simulink model "pmsm_mechanical_bench"  (R2024b)
settings: Solver=ode4  StartTime=0.0  StopTime=bench.StopTime  FixedStep=bench.SolverStep  RelTol=1e-3
model workspace (MAT data in the model file):
  bench.J = 0.002
  bench.B = 0.001
  bench.Tc = 0.02
  bench.FrictionSpeed = 0.2
  bench.QuadraticFriction = 0
  bench.PolePairs = 3
  bench.Flux = 0.03
  bench.Ld = 0.004
  bench.Lq = 0.006
  bench.CurrentTimeConstant = 0.002
  bench.SpeedLoopEnabled = 1
  bench.Kp = 0.2
  bench.Ki = 0.3
  bench.CurrentLimit = 6
  bench.InitialPI = 0
  bench.InitialId = 0
  bench.InitialIq = 0
  bench.InitialSpeed = 35
  bench.SolverStep = 0.0001
  bench.SamplePeriod = 0.001
  bench.StopTime = 3
values from neighbouring files (symbols this model uses):
  bench = struct('Rs',0.7,'Ld',0.004,'Lq',0.006,'Flux',0.03,      'VoltageDrop',0.35,'ResistanceDrop',0.03,'ZeroCurrent',0.15,      'Phase',0,'StopTime',0.6,'SolverStep',1e-5,'SamplePeriod',1e-4,      'InitialDCurrent',0,'InitialQCurrent',0,      'DVoltageBias',1.2,'DVoltageAmplitude',[0.8,0.35],      'DVoltageFrequency',[31,9],'QVoltageBias',5,      'QVoltageAmplitude',[1.1,0.6],'QVoltageFrequency',[17,4], ...(+61 chars)    [pmsm_bench_defaults.m]    (also in pmsm_mechanical_defaults.m = struct('J',0.002,'B',0.001,'Tc',0.02,'FrictionSpeed',0.2,   ; pmsm_run_mechanical_benchmark.m = pmsm_mechanical_defaults(); pmsm_run_simulink_benchmark.m = pmsm_bench_defaults())
settings Model: Creator=lxy  LastModifiedBy=lxy

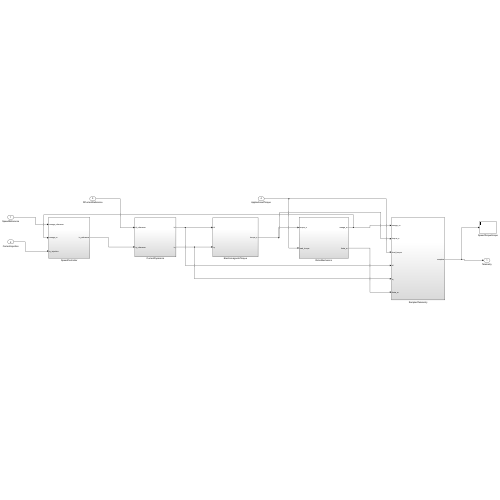
[thumbnail: Simulink's stored preview of the top-level diagram]
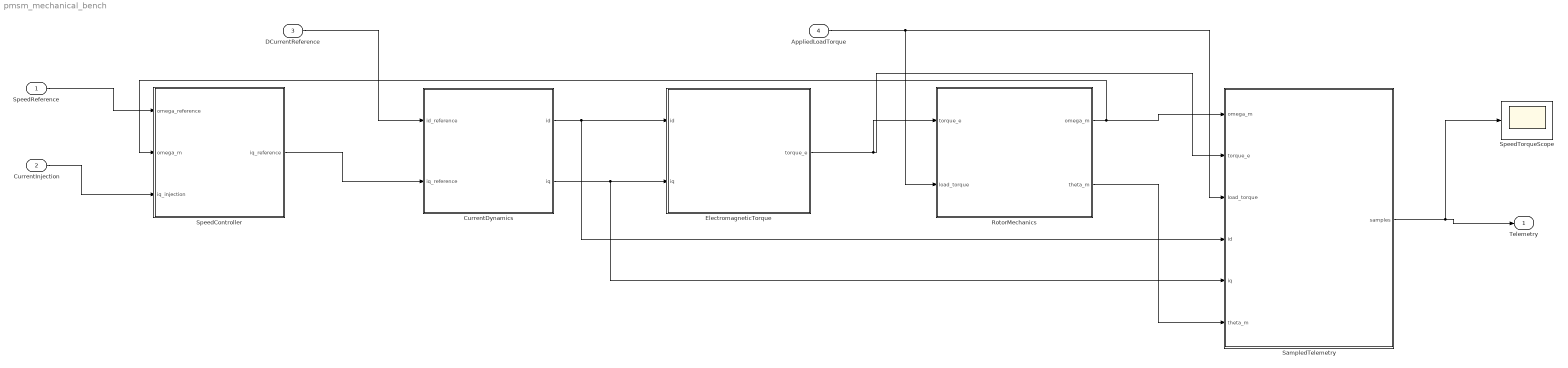
== system pmsm_mechanical_bench ==
  SpeedReference : Inport
  CurrentInjection : Inport  Port=2
  DCurrentReference : Inport  Port=3
  AppliedLoadTorque : Inport  Port=4
  CurrentDynamics : Subsystem
  ElectromagneticTorque : Subsystem
  RotorMechanics : Subsystem
  SampledTelemetry : Subsystem
  SpeedController : Subsystem
  SpeedTorqueScope : Scope
  Telemetry : Outport
  wires:
  SampledTelemetry/1(samples) -> SpeedTorqueScope/1, Telemetry/1
  RotorMechanics/2(theta_m) -> SampledTelemetry/6(theta_m)
  AppliedLoadTorque/1 -> RotorMechanics/2(load_torque), SampledTelemetry/3(load_torque)
  ElectromagneticTorque/1(torque_e) -> SampledTelemetry/2(torque_e), RotorMechanics/1(torque_e)
  CurrentDynamics/2(iq) -> ElectromagneticTorque/2(iq), SampledTelemetry/5(iq)
  CurrentDynamics/1(id) -> ElectromagneticTorque/1(id), SampledTelemetry/4(id)
  SpeedController/1(iq_reference) -> CurrentDynamics/2(iq_reference)
  DCurrentReference/1 -> CurrentDynamics/1(id_reference)
  CurrentInjection/1 -> SpeedController/3(iq_injection)
  RotorMechanics/1(omega_m) -> SpeedController/2(omega_m), SampledTelemetry/1(omega_m)
  SpeedReference/1 -> SpeedController/1(omega_reference)

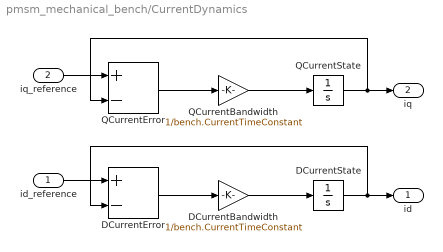
== system pmsm_mechanical_bench/CurrentDynamics ==
  id_reference : Inport
  iq_reference : Inport  Port=2
  DCurrentBandwidth : Gain  Gain=1/bench.CurrentTimeConstant
  DCurrentError : Sum  Inputs=+-
  DCurrentState : Integrator  InitialCondition=bench.InitialId
  QCurrentBandwidth : Gain  Gain=1/bench.CurrentTimeConstant
  QCurrentError : Sum  Inputs=+-
  QCurrentState : Integrator  InitialCondition=bench.InitialIq
  id : Outport
  iq : Outport  Port=2
  wires:
  QCurrentBandwidth/1 -> QCurrentState/1
  QCurrentError/1 -> QCurrentBandwidth/1
  QCurrentState/1 -> QCurrentError/2, iq/1
  iq_reference/1 -> QCurrentError/1
  DCurrentBandwidth/1 -> DCurrentState/1
  DCurrentError/1 -> DCurrentBandwidth/1
  DCurrentState/1 -> DCurrentError/2, id/1
  id_reference/1 -> DCurrentError/1

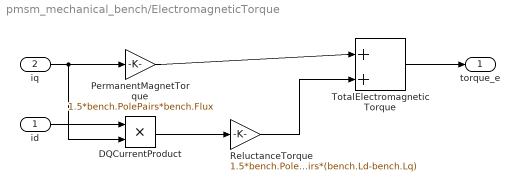
== system pmsm_mechanical_bench/ElectromagneticTorque ==
  id : Inport
  iq : Inport  Port=2
  DQCurrentProduct : Product  Inputs=**
  PermanentMagnetTorque : Gain  Gain=1.5*bench.PolePairs*bench.Flux
  ReluctanceTorque : Gain  Gain=1.5*bench.PolePairs*(bench.Ld-bench.Lq)
  TotalElectromagneticTorque : Sum  Inputs=|++
  torque_e : Outport
  wires:
  TotalElectromagneticTorque/1 -> torque_e/1
  ReluctanceTorque/1 -> TotalElectromagneticTorque/2
  PermanentMagnetTorque/1 -> TotalElectromagneticTorque/1
  DQCurrentProduct/1 -> ReluctanceTorque/1
  id/1 -> DQCurrentProduct/1
  iq/1 -> PermanentMagnetTorque/1, DQCurrentProduct/2

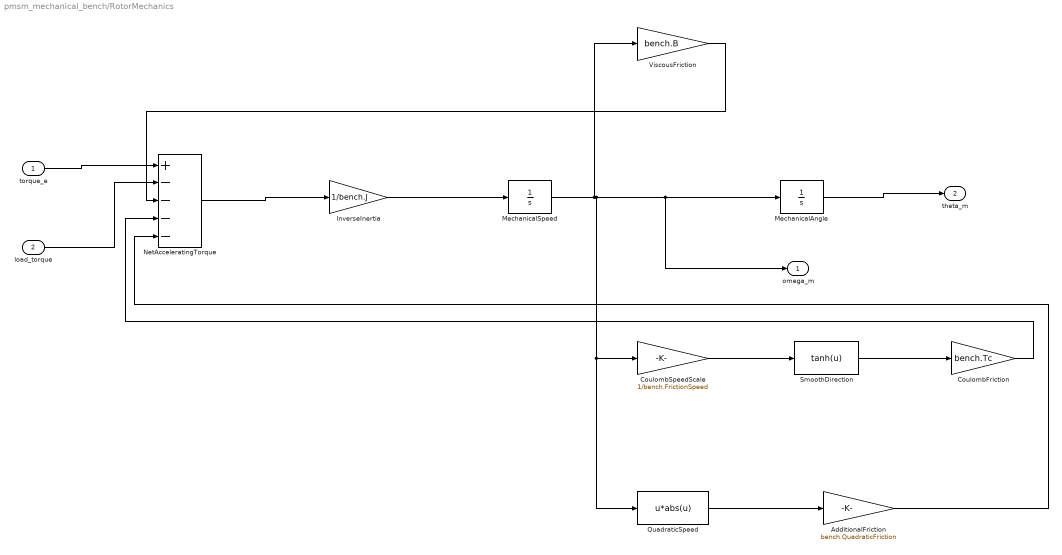
== system pmsm_mechanical_bench/RotorMechanics ==
  torque_e : Inport
  load_torque : Inport  Port=2
  AdditionalFriction : Gain  Gain=bench.QuadraticFriction
  CoulombFriction : Gain  Gain=bench.Tc
  CoulombSpeedScale : Gain  Gain=1/bench.FrictionSpeed
  InverseInertia : Gain  Gain=1/bench.J
  MechanicalAngle : Integrator
  MechanicalSpeed : Integrator  InitialCondition=bench.InitialSpeed
  NetAcceleratingTorque : Sum  Inputs=+----
  QuadraticSpeed : Fcn  Expr=u*abs(u)
  SmoothDirection : Fcn  Expr=tanh(u)
  ViscousFriction : Gain  Gain=bench.B
  omega_m : Outport
  theta_m : Outport  Port=2
  wires:
  MechanicalAngle/1 -> theta_m/1
  QuadraticSpeed/1 -> AdditionalFriction/1
  SmoothDirection/1 -> CoulombFriction/1
  CoulombSpeedScale/1 -> SmoothDirection/1
  MechanicalSpeed/1 -> CoulombSpeedScale/1, QuadraticSpeed/1, omega_m/1, MechanicalAngle/1, ViscousFriction/1
  InverseInertia/1 -> MechanicalSpeed/1
  NetAcceleratingTorque/1 -> InverseInertia/1
  AdditionalFriction/1 -> NetAcceleratingTorque/5
  CoulombFriction/1 -> NetAcceleratingTorque/4
  ViscousFriction/1 -> NetAcceleratingTorque/3
  load_torque/1 -> NetAcceleratingTorque/2
  torque_e/1 -> NetAcceleratingTorque/1

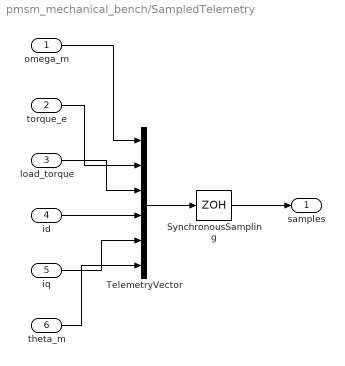
== system pmsm_mechanical_bench/SampledTelemetry ==
  omega_m : Inport
  torque_e : Inport  Port=2
  load_torque : Inport  Port=3
  id : Inport  Port=4
  iq : Inport  Port=5
  theta_m : Inport  Port=6
  SynchronousSampling : ZeroOrderHold  SampleTime=bench.SamplePeriod
  TelemetryVector : Mux  Inputs=6
  samples : Outport
  wires:
  SynchronousSampling/1 -> samples/1
  TelemetryVector/1 -> SynchronousSampling/1
  theta_m/1 -> TelemetryVector/6
  iq/1 -> TelemetryVector/5
  id/1 -> TelemetryVector/4
  load_torque/1 -> TelemetryVector/3
  torque_e/1 -> TelemetryVector/2
  omega_m/1 -> TelemetryVector/1

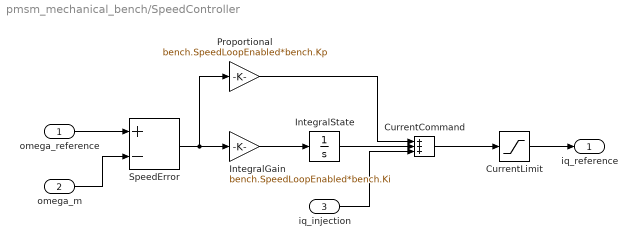
== system pmsm_mechanical_bench/SpeedController ==
  omega_reference : Inport
  omega_m : Inport  Port=2
  iq_injection : Inport  Port=3
  CurrentCommand : Sum  Inputs=+++
  CurrentLimit : Saturate  UpperLimit=bench.CurrentLimit  LowerLimit=-bench.CurrentLimit
  IntegralGain : Gain  Gain=bench.SpeedLoopEnabled*bench.Ki
  IntegralState : Integrator  InitialCondition=bench.InitialPI
  Proportional : Gain  Gain=bench.SpeedLoopEnabled*bench.Kp
  SpeedError : Sum  Inputs=+-
  iq_reference : Outport
  wires:
  CurrentLimit/1 -> iq_reference/1
  CurrentCommand/1 -> CurrentLimit/1
  iq_injection/1 -> CurrentCommand/3
  IntegralState/1 -> CurrentCommand/2
  Proportional/1 -> CurrentCommand/1
  IntegralGain/1 -> IntegralState/1
  SpeedError/1 -> Proportional/1, IntegralGain/1
  omega_m/1 -> SpeedError/2
  omega_reference/1 -> SpeedError/1
